simulink model "ASM_Traffic_A11"  (R2026a)
settings: Solver=ode1  StartTime=SIM.tstart.v  StopTime=SIM.tend.v  FixedStep=SIM.StepSize.v
PostLoadFcn:
  | if any(exist('dsrtsu_mdlpostloadfcn', 'file') ~= 0), dsrtsu_mdlpostloadfcn('Execute', bdroot); end
  | try, asm_mdl_postloadfcn(bdroot, 'UpdateModel', 3600); catch, disp(lasterr); end,
InitFcn:
  | , if any(exist('rtifpga_mdlclblib', 'file') ~= 0), rtifpga_mdlclblib('Init', bdroot); end,
  | , if any(exist('dsmpb_private', 'file') ~= 0), dsmpb_private('dsmpb_mdlclblib', 'Init', bdroot); end,
undefined symbols (not defined in the file): _to_, a0b2, ASM_BrakeHydraulics_DemoSystems, ASM_VehicleDynamics_DemoSystems, b98103fe8ad365046cd0, BrakeCircuit, controllerConfig, CPT, Crankshaft, DiscIntNeverNeededParam, dsmsi, FinalDriveAssembly, instance, MDL, ModeSignals, mu, Pos_BrakePedal_Maneuver, rad, RefSignals, s_to_rpm, SIM, SoftECU, Suspension, Tire, Transmission
libraries: ASM_Traffic_lib x135, simulink x98, ASM_Utils_lib x77, ASM_VehicleDynamics_lib x70, ASM_Environment_lib x22, dsmpblib x20, dsmsilib x15, MDLD_Utils_lib x10, ASM_BrakeHydraulics_lib x3, sl_discontinuities x2
(part 62 of 63)

== system ASM_Traffic_A11/Environment/Sensors/PlantModel/Object_Sensor_3D/ObjectData/Sensor1/Object_Custom_Values/Vectorize_Signals ==
  SensorOutput1 : Inport
  SensorOutput2 : Inport  Port=2
  SensorOutput3 : Inport  Port=3
  Bus Creator : BusCreator  Inputs=2
  Bus Selector : BusSelector  OutputSignals=SensorOutput.Object1.Object_Valid[0|1],SensorOutput.Object2.Object_Valid[0|1],SensorOutput.Object3.Object_Valid[0|1],SensorOutput.Object4.Object_Valid[0|1],SensorOutput.Object5.Object_Valid[0|1]
  Bus Selector1 : BusSelector  OutputSignals=SensorOutput.Object1.Object_Valid[0|1],SensorOutput.Object2.Object_Valid[0|1],SensorOutput.Object3.Object_Valid[0|1],SensorOutput.Object4.Object_Valid[0|1],SensorOutput.Object5.Object_Valid[0|1]
  Bus Selector2 : BusSelector  OutputSignals=SensorOutput.Object1.Object_Valid[0|1],SensorOutput.Object2.Object_Valid[0|1],SensorOutput.Object3.Object_Valid[0|1],SensorOutput.Object4.Object_Valid[0|1],SensorOutput.Object5.Object_Valid[0|1]
  Bus Selector3 : BusSelector  OutputSignals=SensorOutput.Object1.CustomValues[],SensorOutput.Object2.CustomValues[],SensorOutput.Object3.CustomValues[],SensorOutput.Object4.CustomValues[],SensorOutput.Object5.CustomValues[]
  Bus Selector4 : BusSelector  OutputSignals=SensorOutput.Object1.CustomValues[],SensorOutput.Object2.CustomValues[],SensorOutput.Object3.CustomValues[],SensorOutput.Object4.CustomValues[],SensorOutput.Object5.CustomValues[]
  Bus Selector5 : BusSelector  OutputSignals=SensorOutput.Object1.CustomValues[],SensorOutput.Object2.CustomValues[],SensorOutput.Object3.CustomValues[],SensorOutput.Object4.CustomValues[],SensorOutput.Object5.CustomValues[]
  Mux : Mux  Inputs=15
  Mux1 : Mux  Inputs=15
  Vectorized_Custom_Values : Outport  VectorParamsAs1DForOutWhenUnconnected=off
  wires:
  Bus Creator/1 -> Vectorized_Custom_Values/1
  Bus Selector5/5 -> Mux1/15  "<CustomValues[]>"
  Bus Selector5/4 -> Mux1/14  "<CustomValues[]>"
  Bus Selector5/3 -> Mux1/13  "<CustomValues[]>"
  Bus Selector5/2 -> Mux1/12  "<CustomValues[]>"
  Bus Selector5/1 -> Mux1/11  "<CustomValues[]>"
  Bus Selector4/5 -> Mux1/10  "<CustomValues[]>"
  Bus Selector4/4 -> Mux1/9  "<CustomValues[]>"
  Bus Selector4/3 -> Mux1/8  "<CustomValues[]>"
  Bus Selector4/2 -> Mux1/7  "<CustomValues[]>"
  Bus Selector4/1 -> Mux1/6  "<CustomValues[]>"
  Bus Selector3/5 -> Mux1/5  "<CustomValues[]>"
  Bus Selector3/4 -> Mux1/4  "<CustomValues[]>"
  Bus Selector3/3 -> Mux1/3  "<CustomValues[]>"
  Bus Selector3/2 -> Mux1/2  "<CustomValues[]>"
  Bus Selector3/1 -> Mux1/1  "<CustomValues[]>"
  Bus Selector2/5 -> Mux/15  "<Object_Valid[0|1]>"
  Bus Selector2/4 -> Mux/14  "<Object_Valid[0|1]>"
  Bus Selector2/3 -> Mux/13  "<Object_Valid[0|1]>"
  Bus Selector2/2 -> Mux/12  "<Object_Valid[0|1]>"
  Bus Selector2/1 -> Mux/11  "<Object_Valid[0|1]>"
  Bus Selector1/5 -> Mux/10  "<Object_Valid[0|1]>"
  Bus Selector1/4 -> Mux/9  "<Object_Valid[0|1]>"
  Bus Selector1/3 -> Mux/8  "<Object_Valid[0|1]>"
  Bus Selector1/2 -> Mux/7  "<Object_Valid[0|1]>"
  Bus Selector1/1 -> Mux/6  "<Object_Valid[0|1]>"
  Mux1/1 -> Bus Creator/2  "CustomValues[]"
  Mux/1 -> Bus Creator/1  "Object_Valid[0|1]"
  SensorOutput3/1 -> Bus Selector2/1, Bus Selector5/1
  SensorOutput2/1 -> Bus Selector1/1, Bus Selector4/1
  Bus Selector/1 -> Mux/1  "<Object_Valid[0|1]>"
  Bus Selector/2 -> Mux/2  "<Object_Valid[0|1]>"
  Bus Selector/3 -> Mux/3  "<Object_Valid[0|1]>"
  Bus Selector/4 -> Mux/4  "<Object_Valid[0|1]>"
  Bus Selector/5 -> Mux/5  "<Object_Valid[0|1]>"
  SensorOutput1/1 -> Bus Selector3/1, Bus Selector/1

== system ASM_Traffic_A11/Environment/Sensors/PlantModel/Object_Sensor_3D/ObjectData/Sensor2/Object_Custom_Values/Vectorize_Signals ==
  SensorOutput1 : Inport
  SensorOutput2 : Inport  Port=2
  SensorOutput3 : Inport  Port=3
  Bus Creator : BusCreator  Inputs=2
  Bus Selector : BusSelector  OutputSignals=SensorOutput.Object1.Object_Valid[0|1],SensorOutput.Object2.Object_Valid[0|1],SensorOutput.Object3.Object_Valid[0|1],SensorOutput.Object4.Object_Valid[0|1],SensorOutput.Object5.Object_Valid[0|1]
  Bus Selector1 : BusSelector  OutputSignals=SensorOutput.Object1.Object_Valid[0|1],SensorOutput.Object2.Object_Valid[0|1],SensorOutput.Object3.Object_Valid[0|1],SensorOutput.Object4.Object_Valid[0|1],SensorOutput.Object5.Object_Valid[0|1]
  Bus Selector2 : BusSelector  OutputSignals=SensorOutput.Object1.Object_Valid[0|1],SensorOutput.Object2.Object_Valid[0|1],SensorOutput.Object3.Object_Valid[0|1],SensorOutput.Object4.Object_Valid[0|1],SensorOutput.Object5.Object_Valid[0|1]
  Bus Selector3 : BusSelector  OutputSignals=SensorOutput.Object1.CustomValues[],SensorOutput.Object2.CustomValues[],SensorOutput.Object3.CustomValues[],SensorOutput.Object4.CustomValues[],SensorOutput.Object5.CustomValues[]
  Bus Selector4 : BusSelector  OutputSignals=SensorOutput.Object1.CustomValues[],SensorOutput.Object2.CustomValues[],SensorOutput.Object3.CustomValues[],SensorOutput.Object4.CustomValues[],SensorOutput.Object5.CustomValues[]
  Bus Selector5 : BusSelector  OutputSignals=SensorOutput.Object1.CustomValues[],SensorOutput.Object2.CustomValues[],SensorOutput.Object3.CustomValues[],SensorOutput.Object4.CustomValues[],SensorOutput.Object5.CustomValues[]
  Mux : Mux  Inputs=15
  Mux1 : Mux  Inputs=15
  Vectorized_Custom_Values : Outport  VectorParamsAs1DForOutWhenUnconnected=off
  wires:
  SensorOutput1/1 -> Bus Selector/1, Bus Selector3/1
  Bus Selector/5 -> Mux/5  "<Object_Valid[0|1]>"
  Bus Selector/4 -> Mux/4  "<Object_Valid[0|1]>"
  Bus Selector/3 -> Mux/3  "<Object_Valid[0|1]>"
  Bus Selector/2 -> Mux/2  "<Object_Valid[0|1]>"
  Bus Selector/1 -> Mux/1  "<Object_Valid[0|1]>"
  SensorOutput2/1 -> Bus Selector4/1, Bus Selector1/1
  SensorOutput3/1 -> Bus Selector5/1, Bus Selector2/1
  Mux/1 -> Bus Creator/1  "Object_Valid[0|1]"
  Mux1/1 -> Bus Creator/2  "CustomValues[]"
  Bus Selector1/1 -> Mux/6  "<Object_Valid[0|1]>"
  Bus Selector1/2 -> Mux/7  "<Object_Valid[0|1]>"
  Bus Selector1/3 -> Mux/8  "<Object_Valid[0|1]>"
  Bus Selector1/4 -> Mux/9  "<Object_Valid[0|1]>"
  Bus Selector1/5 -> Mux/10  "<Object_Valid[0|1]>"
  Bus Selector2/1 -> Mux/11  "<Object_Valid[0|1]>"
  Bus Selector2/2 -> Mux/12  "<Object_Valid[0|1]>"
  Bus Selector2/3 -> Mux/13  "<Object_Valid[0|1]>"
  Bus Selector2/4 -> Mux/14  "<Object_Valid[0|1]>"
  Bus Selector2/5 -> Mux/15  "<Object_Valid[0|1]>"
  Bus Selector3/1 -> Mux1/1  "<CustomValues[]>"
  Bus Selector3/2 -> Mux1/2  "<CustomValues[]>"
  Bus Selector3/3 -> Mux1/3  "<CustomValues[]>"
  Bus Selector3/4 -> Mux1/4  "<CustomValues[]>"
  Bus Selector3/5 -> Mux1/5  "<CustomValues[]>"
  Bus Selector4/1 -> Mux1/6  "<CustomValues[]>"
  Bus Selector4/2 -> Mux1/7  "<CustomValues[]>"
  Bus Selector4/3 -> Mux1/8  "<CustomValues[]>"
  Bus Selector4/4 -> Mux1/9  "<CustomValues[]>"
  Bus Selector4/5 -> Mux1/10  "<CustomValues[]>"
  Bus Selector5/1 -> Mux1/11  "<CustomValues[]>"
  Bus Selector5/2 -> Mux1/12  "<CustomValues[]>"
  Bus Selector5/3 -> Mux1/13  "<CustomValues[]>"
  Bus Selector5/4 -> Mux1/14  "<CustomValues[]>"
  Bus Selector5/5 -> Mux1/15  "<CustomValues[]>"
  Bus Creator/1 -> Vectorized_Custom_Values/1

== system ASM_Traffic_A11/Environment/Sensors/PlantModel/Object_Sensor_3D/ObjectData/Sensor3/Object_Custom_Values/Vectorize_Signals ==
  SensorOutput1 : Inport
  SensorOutput2 : Inport  Port=2
  SensorOutput3 : Inport  Port=3
  Bus Creator : BusCreator  Inputs=2
  Bus Selector : BusSelector  OutputSignals=SensorOutput.Object1.Object_Valid[0|1],SensorOutput.Object2.Object_Valid[0|1],SensorOutput.Object3.Object_Valid[0|1],SensorOutput.Object4.Object_Valid[0|1],SensorOutput.Object5.Object_Valid[0|1]
  Bus Selector1 : BusSelector  OutputSignals=SensorOutput.Object1.Object_Valid[0|1],SensorOutput.Object2.Object_Valid[0|1],SensorOutput.Object3.Object_Valid[0|1],SensorOutput.Object4.Object_Valid[0|1],SensorOutput.Object5.Object_Valid[0|1]
  Bus Selector2 : BusSelector  OutputSignals=SensorOutput.Object1.Object_Valid[0|1],SensorOutput.Object2.Object_Valid[0|1],SensorOutput.Object3.Object_Valid[0|1],SensorOutput.Object4.Object_Valid[0|1],SensorOutput.Object5.Object_Valid[0|1]
  Bus Selector3 : BusSelector  OutputSignals=SensorOutput.Object1.CustomValues[],SensorOutput.Object2.CustomValues[],SensorOutput.Object3.CustomValues[],SensorOutput.Object4.CustomValues[],SensorOutput.Object5.CustomValues[]
  Bus Selector4 : BusSelector  OutputSignals=SensorOutput.Object1.CustomValues[],SensorOutput.Object2.CustomValues[],SensorOutput.Object3.CustomValues[],SensorOutput.Object4.CustomValues[],SensorOutput.Object5.CustomValues[]
  Bus Selector5 : BusSelector  OutputSignals=SensorOutput.Object1.CustomValues[],SensorOutput.Object2.CustomValues[],SensorOutput.Object3.CustomValues[],SensorOutput.Object4.CustomValues[],SensorOutput.Object5.CustomValues[]
  Mux : Mux  Inputs=15
  Mux1 : Mux  Inputs=15
  Vectorized_Custom_Values : Outport  VectorParamsAs1DForOutWhenUnconnected=off
  wires:
  Bus Creator/1 -> Vectorized_Custom_Values/1
  Bus Selector5/5 -> Mux1/15  "<CustomValues[]>"
  Bus Selector5/4 -> Mux1/14  "<CustomValues[]>"
  Bus Selector5/3 -> Mux1/13  "<CustomValues[]>"
  Bus Selector5/2 -> Mux1/12  "<CustomValues[]>"
  Bus Selector5/1 -> Mux1/11  "<CustomValues[]>"
  Bus Selector4/5 -> Mux1/10  "<CustomValues[]>"
  Bus Selector4/4 -> Mux1/9  "<CustomValues[]>"
  Bus Selector4/3 -> Mux1/8  "<CustomValues[]>"
  Bus Selector4/2 -> Mux1/7  "<CustomValues[]>"
  Bus Selector4/1 -> Mux1/6  "<CustomValues[]>"
  Bus Selector3/5 -> Mux1/5  "<CustomValues[]>"
  Bus Selector3/4 -> Mux1/4  "<CustomValues[]>"
  Bus Selector3/3 -> Mux1/3  "<CustomValues[]>"
  Bus Selector3/2 -> Mux1/2  "<CustomValues[]>"
  Bus Selector3/1 -> Mux1/1  "<CustomValues[]>"
  Bus Selector2/5 -> Mux/15  "<Object_Valid[0|1]>"
  Bus Selector2/4 -> Mux/14  "<Object_Valid[0|1]>"
  Bus Selector2/3 -> Mux/13  "<Object_Valid[0|1]>"
  Bus Selector2/2 -> Mux/12  "<Object_Valid[0|1]>"
  Bus Selector2/1 -> Mux/11  "<Object_Valid[0|1]>"
  Bus Selector1/5 -> Mux/10  "<Object_Valid[0|1]>"
  Bus Selector1/4 -> Mux/9  "<Object_Valid[0|1]>"
  Bus Selector1/3 -> Mux/8  "<Object_Valid[0|1]>"
  Bus Selector1/2 -> Mux/7  "<Object_Valid[0|1]>"
  Bus Selector1/1 -> Mux/6  "<Object_Valid[0|1]>"
  Mux1/1 -> Bus Creator/2  "CustomValues[]"
  Mux/1 -> Bus Creator/1  "Object_Valid[0|1]"
  SensorOutput3/1 -> Bus Selector2/1, Bus Selector5/1
  SensorOutput2/1 -> Bus Selector1/1, Bus Selector4/1
  Bus Selector/1 -> Mux/1  "<Object_Valid[0|1]>"
  Bus Selector/2 -> Mux/2  "<Object_Valid[0|1]>"
  Bus Selector/3 -> Mux/3  "<Object_Valid[0|1]>"
  Bus Selector/4 -> Mux/4  "<Object_Valid[0|1]>"
  Bus Selector/5 -> Mux/5  "<Object_Valid[0|1]>"
  SensorOutput1/1 -> Bus Selector3/1, Bus Selector/1

== system ASM_Traffic_A11/Environment/Sensors/PlantModel/Object_Sensor_3D/RadarEffects/Sensor1/RadarEffectsOutput/HoldSignals ==
  ResetPulse[0|1] : Inport
  RadarEffect_Signals_In[] : Inport  Port=2
  Enable : EnablePort
  Bus Selector1 : BusSelector  OutputSignals=ID[],Dist_CoorSys_S[m],v_CoorSys_S[m|s],Angle_Hor_CoorSys_S[deg],Angle_Ver_CoorSys_S[deg],RCS[dBm2],Object_ID[],Object_Type[],Pos_ObjectPoint_CoorSys_E[x;y;z][m],Pos_ObjectPoint_CoorSys_S[x;y;z][m]
  RADAR_SIGNALS_RESET_1 : ASM_Traffic_lib/Sensors/RadarEffects/RADAR_SIGNALS_RESET  ASMProperties=struct('Name','RADAR_SIGNALS_RESET','Version','1.0','Library','ASM_Traffic_lib')  ASMInstanceName=radar_signals_reset  ASMInstanceID=1
  RadarEffect_Signals_Out[] : Outport  VectorParamsAs1DForOutWhenUnconnected=off
  wires:
  ResetPulse[0|1]/1 -> RADAR_SIGNALS_RESET_1/1
  RADAR_SIGNALS_RESET_1/1 -> RadarEffect_Signals_Out[]/1
  Bus Selector1/3 -> RADAR_SIGNALS_RESET_1/4  "<v_CoorSys_S[m|s]>"
  Bus Selector1/2 -> RADAR_SIGNALS_RESET_1/3  "<Dist_CoorSys_S[m]>"
  Bus Selector1/7 -> RADAR_SIGNALS_RESET_1/8  "<Object_ID[]>"
  Bus Selector1/6 -> RADAR_SIGNALS_RESET_1/7  "<RCS[dBm2]>"
  Bus Selector1/4 -> RADAR_SIGNALS_RESET_1/5  "<Angle_Hor_CoorSys_S[deg]>"
  Bus Selector1/1 -> RADAR_SIGNALS_RESET_1/2  "<ID[]>"
  Bus Selector1/9 -> RADAR_SIGNALS_RESET_1/10  "<Pos_ObjectPoint_CoorSys_E[x;y;z][m]>"
  Bus Selector1/5 -> RADAR_SIGNALS_RESET_1/6  "<Angle_Ver_CoorSys_S[deg]>"
  Bus Selector1/8 -> RADAR_SIGNALS_RESET_1/9  "<Object_Type[]>"
  Bus Selector1/10 -> RADAR_SIGNALS_RESET_1/11  "<Pos_ObjectPoint_CoorSys_S[x;y;z][m]>"
  RadarEffect_Signals_In[]/1 -> Bus Selector1/1

== system ASM_Traffic_A11/Environment/Sensors/PlantModel/Object_Sensor_3D/RadarEffects/Sensor1/RadarEffectsOutput/ResetPulse ==
  Enable[0|1] : Inport
  SensorActive[0|1] : Inport  Port=2
  Compare To Constant : simulink/Logic and Bit Operations/Compare To Constant  relop===  const=1  OutDataTypeStr=boolean
  Compare To Constant1 : simulink/Logic and Bit Operations/Compare To Constant  relop===  const=0  OutDataTypeStr=boolean
  Logical Operator1 : Logic  AllPortsSameDT=off  OutDataTypeStr=boolean
  Logical Operator2 : Logic  Operator=NAND  AllPortsSameDT=off  OutDataTypeStr=boolean
  Memory1 : UnitDelay  SampleTime=-1
  ResetPulse[0|1] : Outport  VectorParamsAs1DForOutWhenUnconnected=off
  wires:
  Memory1/1 -> Compare To Constant1/1
  Logical Operator2/1 -> Compare To Constant/1, Memory1/1
  SensorActive[0|1]/1 -> Logical Operator2/1
  Logical Operator1/1 -> ResetPulse[0|1]/1
  Compare To Constant/1 -> Logical Operator1/1
  Compare To Constant1/1 -> Logical Operator1/2
  Enable[0|1]/1 -> Logical Operator2/2

== system ASM_Traffic_A11/Environment/Sensors/PlantModel/Object_Sensor_3D/RadarEffects/Sensor1/RadarEffectsOutput/SignalBus ==
  RadarEffect_Signals_In[] : Inport
  Bus Creator : BusCreator  Inputs=5
  Bus Selector1 : BusSelector  OutputSignals=ID[],Object_ID[],Dist_CoorSys_S[m],Angle_Hor_CoorSys_S[deg],Pos_ObjectPoint_CoorSys_E[x;y;z][m]
  RadarEffect_Signals_Out[] : Outport  VectorParamsAs1DForOutWhenUnconnected=off
  wires:
  RadarEffect_Signals_In[]/1 -> Bus Selector1/1
  Bus Creator/1 -> RadarEffect_Signals_Out[]/1
  Bus Selector1/4 -> Bus Creator/4  "<Angle_Hor_CoorSys_S[deg]>"
  Bus Selector1/5 -> Bus Creator/5  "<Pos_ObjectPoint_CoorSys_E[x;y;z][m]>"
  Bus Selector1/2 -> Bus Creator/2  "<Object_ID[]>"
  Bus Selector1/3 -> Bus Creator/3  "<Dist_CoorSys_S[m]>"
  Bus Selector1/1 -> Bus Creator/1  "<ID[]>"

== system ASM_Traffic_A11/Environment/Sensors/PlantModel/Object_Sensor_3D/RadarEffects/Sensor2/RadarEffectsOutput/HoldSignals ==
  ResetPulse[0|1] : Inport
  RadarEffect_Signals_In[] : Inport  Port=2
  Enable : EnablePort
  Bus Selector1 : BusSelector  OutputSignals=ID[],Dist_CoorSys_S[m],v_CoorSys_S[m|s],Angle_Hor_CoorSys_S[deg],Angle_Ver_CoorSys_S[deg],RCS[dBm2],Object_ID[],Object_Type[],Pos_ObjectPoint_CoorSys_E[x;y;z][m],Pos_ObjectPoint_CoorSys_S[x;y;z][m]
  RADAR_SIGNALS_RESET_2 : ASM_Traffic_lib/Sensors/RadarEffects/RADAR_SIGNALS_RESET  ASMProperties=struct('Name','RADAR_SIGNALS_RESET','Version','1.0','Library','ASM_Traffic_lib')  ASMInstanceName=radar_signals_reset  ASMInstanceID=1
  RadarEffect_Signals_Out[] : Outport  VectorParamsAs1DForOutWhenUnconnected=off
  wires:
  ResetPulse[0|1]/1 -> RADAR_SIGNALS_RESET_2/1
  Bus Selector1/8 -> RADAR_SIGNALS_RESET_2/9  "<Object_Type[]>"
  Bus Selector1/3 -> RADAR_SIGNALS_RESET_2/4  "<v_CoorSys_S[m|s]>"
  Bus Selector1/7 -> RADAR_SIGNALS_RESET_2/8  "<Object_ID[]>"
  RadarEffect_Signals_In[]/1 -> Bus Selector1/1
  Bus Selector1/6 -> RADAR_SIGNALS_RESET_2/7  "<RCS[dBm2]>"
  Bus Selector1/5 -> RADAR_SIGNALS_RESET_2/6  "<Angle_Ver_CoorSys_S[deg]>"
  Bus Selector1/4 -> RADAR_SIGNALS_RESET_2/5  "<Angle_Hor_CoorSys_S[deg]>"
  Bus Selector1/2 -> RADAR_SIGNALS_RESET_2/3  "<Dist_CoorSys_S[m]>"
  Bus Selector1/10 -> RADAR_SIGNALS_RESET_2/11  "<Pos_ObjectPoint_CoorSys_S[x;y;z][m]>"
  Bus Selector1/1 -> RADAR_SIGNALS_RESET_2/2  "<ID[]>"
  Bus Selector1/9 -> RADAR_SIGNALS_RESET_2/10  "<Pos_ObjectPoint_CoorSys_E[x;y;z][m]>"
  RADAR_SIGNALS_RESET_2/1 -> RadarEffect_Signals_Out[]/1

== system ASM_Traffic_A11/Environment/Sensors/PlantModel/Object_Sensor_3D/RadarEffects/Sensor2/RadarEffectsOutput/ResetPulse ==
  Enable[0|1] : Inport
  SensorActive[0|1] : Inport  Port=2
  Compare To Constant : simulink/Logic and Bit Operations/Compare To Constant  relop===  const=1  OutDataTypeStr=boolean
  Compare To Constant1 : simulink/Logic and Bit Operations/Compare To Constant  relop===  const=0  OutDataTypeStr=boolean
  Logical Operator1 : Logic  AllPortsSameDT=off  OutDataTypeStr=boolean
  Logical Operator2 : Logic  Operator=NAND  AllPortsSameDT=off  OutDataTypeStr=boolean
  Memory1 : UnitDelay  SampleTime=-1
  ResetPulse[0|1] : Outport  VectorParamsAs1DForOutWhenUnconnected=off
  wires:
  Memory1/1 -> Compare To Constant1/1
  Logical Operator2/1 -> Compare To Constant/1, Memory1/1
  SensorActive[0|1]/1 -> Logical Operator2/1
  Logical Operator1/1 -> ResetPulse[0|1]/1
  Compare To Constant/1 -> Logical Operator1/1
  Compare To Constant1/1 -> Logical Operator1/2
  Enable[0|1]/1 -> Logical Operator2/2

== system ASM_Traffic_A11/Environment/Sensors/PlantModel/Object_Sensor_3D/RadarEffects/Sensor2/RadarEffectsOutput/SignalBus ==
  RadarEffect_Signals_In[] : Inport
  Bus Creator : BusCreator  Inputs=5
  Bus Selector1 : BusSelector  OutputSignals=ID[],Object_ID[],Dist_CoorSys_S[m],Angle_Hor_CoorSys_S[deg],Pos_ObjectPoint_CoorSys_E[x;y;z][m]
  RadarEffect_Signals_Out[] : Outport  VectorParamsAs1DForOutWhenUnconnected=off
  wires:
  RadarEffect_Signals_In[]/1 -> Bus Selector1/1
  Bus Creator/1 -> RadarEffect_Signals_Out[]/1
  Bus Selector1/4 -> Bus Creator/4  "<Angle_Hor_CoorSys_S[deg]>"
  Bus Selector1/5 -> Bus Creator/5  "<Pos_ObjectPoint_CoorSys_E[x;y;z][m]>"
  Bus Selector1/2 -> Bus Creator/2  "<Object_ID[]>"
  Bus Selector1/3 -> Bus Creator/3  "<Dist_CoorSys_S[m]>"
  Bus Selector1/1 -> Bus Creator/1  "<ID[]>"

== system ASM_Traffic_A11/Environment/Sensors/PlantModel/Object_Sensor_3D/RadarEffects/Sensor3/RadarEffectsOutput/HoldSignals ==
  ResetPulse[0|1] : Inport
  RadarEffect_Signals_In[] : Inport  Port=2
  Enable : EnablePort
  Bus Selector1 : BusSelector  OutputSignals=ID[],Dist_CoorSys_S[m],v_CoorSys_S[m|s],Angle_Hor_CoorSys_S[deg],Angle_Ver_CoorSys_S[deg],RCS[dBm2],Object_ID[],Object_Type[],Pos_ObjectPoint_CoorSys_E[x;y;z][m],Pos_ObjectPoint_CoorSys_S[x;y;z][m]
  RADAR_SIGNALS_RESET_3 : ASM_Traffic_lib/Sensors/RadarEffects/RADAR_SIGNALS_RESET  ASMProperties=struct('Name','RADAR_SIGNALS_RESET','Version','1.0','Library','ASM_Traffic_lib')  ASMInstanceName=radar_signals_reset  ASMInstanceID=1
  RadarEffect_Signals_Out[] : Outport  VectorParamsAs1DForOutWhenUnconnected=off
  wires:
  RADAR_SIGNALS_RESET_3/1 -> RadarEffect_Signals_Out[]/1
  Bus Selector1/9 -> RADAR_SIGNALS_RESET_3/10  "<Pos_ObjectPoint_CoorSys_E[x;y;z][m]>"
  Bus Selector1/5 -> RADAR_SIGNALS_RESET_3/6  "<Angle_Ver_CoorSys_S[deg]>"
  Bus Selector1/4 -> RADAR_SIGNALS_RESET_3/5  "<Angle_Hor_CoorSys_S[deg]>"
  Bus Selector1/1 -> RADAR_SIGNALS_RESET_3/2  "<ID[]>"
  ResetPulse[0|1]/1 -> RADAR_SIGNALS_RESET_3/1
  Bus Selector1/6 -> RADAR_SIGNALS_RESET_3/7  "<RCS[dBm2]>"
  Bus Selector1/7 -> RADAR_SIGNALS_RESET_3/8  "<Object_ID[]>"
  Bus Selector1/3 -> RADAR_SIGNALS_RESET_3/4  "<v_CoorSys_S[m|s]>"
  RadarEffect_Signals_In[]/1 -> Bus Selector1/1
  Bus Selector1/10 -> RADAR_SIGNALS_RESET_3/11  "<Pos_ObjectPoint_CoorSys_S[x;y;z][m]>"
  Bus Selector1/8 -> RADAR_SIGNALS_RESET_3/9  "<Object_Type[]>"
  Bus Selector1/2 -> RADAR_SIGNALS_RESET_3/3  "<Dist_CoorSys_S[m]>"

== system ASM_Traffic_A11/Environment/Sensors/PlantModel/Object_Sensor_3D/RadarEffects/Sensor3/RadarEffectsOutput/ResetPulse ==
  Enable[0|1] : Inport
  SensorActive[0|1] : Inport  Port=2
  Compare To Constant : simulink/Logic and Bit Operations/Compare To Constant  relop===  const=1  OutDataTypeStr=boolean
  Compare To Constant1 : simulink/Logic and Bit Operations/Compare To Constant  relop===  const=0  OutDataTypeStr=boolean
  Logical Operator1 : Logic  AllPortsSameDT=off  OutDataTypeStr=boolean
  Logical Operator2 : Logic  Operator=NAND  AllPortsSameDT=off  OutDataTypeStr=boolean
  Memory1 : UnitDelay  SampleTime=-1
  ResetPulse[0|1] : Outport  VectorParamsAs1DForOutWhenUnconnected=off
  wires:
  Memory1/1 -> Compare To Constant1/1
  Logical Operator2/1 -> Compare To Constant/1, Memory1/1
  SensorActive[0|1]/1 -> Logical Operator2/1
  Logical Operator1/1 -> ResetPulse[0|1]/1
  Compare To Constant/1 -> Logical Operator1/1
  Compare To Constant1/1 -> Logical Operator1/2
  Enable[0|1]/1 -> Logical Operator2/2

== system ASM_Traffic_A11/Environment/Sensors/PlantModel/Object_Sensor_3D/RadarEffects/Sensor3/RadarEffectsOutput/SignalBus ==
  RadarEffect_Signals_In[] : Inport
  Bus Creator : BusCreator  Inputs=5
  Bus Selector1 : BusSelector  OutputSignals=ID[],Object_ID[],Dist_CoorSys_S[m],Angle_Hor_CoorSys_S[deg],Pos_ObjectPoint_CoorSys_E[x;y;z][m]
  RadarEffect_Signals_Out[] : Outport  VectorParamsAs1DForOutWhenUnconnected=off
  wires:
  RadarEffect_Signals_In[]/1 -> Bus Selector1/1
  Bus Creator/1 -> RadarEffect_Signals_Out[]/1
  Bus Selector1/4 -> Bus Creator/4  "<Angle_Hor_CoorSys_S[deg]>"
  Bus Selector1/5 -> Bus Creator/5  "<Pos_ObjectPoint_CoorSys_E[x;y;z][m]>"
  Bus Selector1/2 -> Bus Creator/2  "<Object_ID[]>"
  Bus Selector1/3 -> Bus Creator/3  "<Dist_CoorSys_S[m]>"
  Bus Selector1/1 -> Bus Creator/1  "<ID[]>"

== system ASM_Traffic_A11/Environment/Sensors/UserInterface/DISP_Plant/Object_Sensor_2D/IdxSelect_2DSensor/Scopezone_Element_Data_Selection1/Angle_Hor_Rel[deg]1 ==
  In1 : Inport
  Out1 : Outport  VectorParamsAs1DForOutWhenUnconnected=off
  wires:
  In1/1 -> Out1/1

== system ASM_Traffic_A11/Environment/Sensors/UserInterface/DISP_Plant/Object_Sensor_2D/IdxSelect_2DSensor/Scopezone_Element_Data_Selection1/Distance[m]1 ==
  In1 : Inport
  Out1 : Outport  VectorParamsAs1DForOutWhenUnconnected=off
  wires:
  In1/1 -> Out1/1

== system ASM_Traffic_A11/Environment/Sensors/UserInterface/DISP_Plant/Object_Sensor_2D/IdxSelect_2DSensor/Scopezone_Element_Data_Selection1/Flag_Object_In_Scope[0Out|1In]1 ==
  In1 : Inport
  Out1 : Outport  VectorParamsAs1DForOutWhenUnconnected=off
  wires:
  In1/1 -> Out1/1

== system ASM_Traffic_A11/Environment/Sensors/UserInterface/DISP_Plant/Object_Sensor_2D/IdxSelect_2DSensor/Scopezone_Element_Data_Selection1/Flag_Sensor_Apex_In_Object[0Out|1In]1 ==
  In1 : Inport
  Out1 : Outport  VectorParamsAs1DForOutWhenUnconnected=off
  wires:
  In1/1 -> Out1/1

== system ASM_Traffic_A11/Environment/Sensors/UserInterface/DISP_Plant/Object_Sensor_2D/IdxSelect_2DSensor/Scopezone_Element_Data_Selection1/Height_Max[m]1 ==
  In1 : Inport
  Out1 : Outport  VectorParamsAs1DForOutWhenUnconnected=off
  wires:
  In1/1 -> Out1/1

== system ASM_Traffic_A11/Environment/Sensors/UserInterface/DISP_Plant/Object_Sensor_2D/IdxSelect_2DSensor/Scopezone_Element_Data_Selection1/Height_Min[m]1 ==
  In1 : Inport
  Out1 : Outport  VectorParamsAs1DForOutWhenUnconnected=off
  wires:
  In1/1 -> Out1/1

== system ASM_Traffic_A11/Environment/Sensors/UserInterface/DISP_Plant/Object_Sensor_2D/IdxSelect_2DSensor/Scopezone_Element_Data_Selection1/Object_ID[]1 ==
  In1 : Inport
  Out1 : Outport  VectorParamsAs1DForOutWhenUnconnected=off
  wires:
  In1/1 -> Out1/1

== system ASM_Traffic_A11/Environment/Sensors/UserInterface/DISP_Plant/Object_Sensor_2D/IdxSelect_2DSensor/Scopezone_Element_Data_Selection1/Object_Type[]1 ==
  In1 : Inport
  Out1 : Outport  VectorParamsAs1DForOutWhenUnconnected=off
  wires:
  In1/1 -> Out1/1

== system ASM_Traffic_A11/Environment/Sensors/UserInterface/DISP_Plant/Object_Sensor_2D/IdxSelect_2DSensor/Scopezone_Element_Data_Selection1/a_Rel[m|s2]1 ==
  In1 : Inport
  Out1 : Outport  VectorParamsAs1DForOutWhenUnconnected=off
  wires:
  In1/1 -> Out1/1

== system ASM_Traffic_A11/Environment/Sensors/UserInterface/DISP_Plant/Object_Sensor_2D/IdxSelect_2DSensor/Scopezone_Element_Data_Selection1/v_Rel[m|s]1 ==
  In1 : Inport
  Out1 : Outport  VectorParamsAs1DForOutWhenUnconnected=off
  wires:
  In1/1 -> Out1/1

== system ASM_Traffic_A11/Environment/Sensors/UserInterface/DISP_Plant/Object_Sensor_2D/IdxSelect_2DSensor/Scopezone_Element_Data_Selection2/Angle_Hor_Rel[deg]1 ==
  In1 : Inport
  Out1 : Outport  VectorParamsAs1DForOutWhenUnconnected=off
  wires:
  In1/1 -> Out1/1

== system ASM_Traffic_A11/Environment/Sensors/UserInterface/DISP_Plant/Object_Sensor_2D/IdxSelect_2DSensor/Scopezone_Element_Data_Selection2/Distance[m]1 ==
  In1 : Inport
  Out1 : Outport  VectorParamsAs1DForOutWhenUnconnected=off
  wires:
  In1/1 -> Out1/1

== system ASM_Traffic_A11/Environment/Sensors/UserInterface/DISP_Plant/Object_Sensor_2D/IdxSelect_2DSensor/Scopezone_Element_Data_Selection2/Flag_Object_In_Scope[0Out|1In]1 ==
  In1 : Inport
  Out1 : Outport  VectorParamsAs1DForOutWhenUnconnected=off
  wires:
  In1/1 -> Out1/1

== system ASM_Traffic_A11/Environment/Sensors/UserInterface/DISP_Plant/Object_Sensor_2D/IdxSelect_2DSensor/Scopezone_Element_Data_Selection2/Flag_Sensor_Apex_In_Object[0Out|1In]1 ==
  In1 : Inport
  Out1 : Outport  VectorParamsAs1DForOutWhenUnconnected=off
  wires:
  In1/1 -> Out1/1

== system ASM_Traffic_A11/Environment/Sensors/UserInterface/DISP_Plant/Object_Sensor_2D/IdxSelect_2DSensor/Scopezone_Element_Data_Selection2/Height_Max[m]1 ==
  In1 : Inport
  Out1 : Outport  VectorParamsAs1DForOutWhenUnconnected=off
  wires:
  In1/1 -> Out1/1

== system ASM_Traffic_A11/Environment/Sensors/UserInterface/DISP_Plant/Object_Sensor_2D/IdxSelect_2DSensor/Scopezone_Element_Data_Selection2/Height_Min[m]1 ==
  In1 : Inport
  Out1 : Outport  VectorParamsAs1DForOutWhenUnconnected=off
  wires:
  In1/1 -> Out1/1

== system ASM_Traffic_A11/Environment/Sensors/UserInterface/DISP_Plant/Object_Sensor_2D/IdxSelect_2DSensor/Scopezone_Element_Data_Selection2/Object_ID[]1 ==
  In1 : Inport
  Out1 : Outport  VectorParamsAs1DForOutWhenUnconnected=off
  wires:
  In1/1 -> Out1/1

== system ASM_Traffic_A11/Environment/Sensors/UserInterface/DISP_Plant/Object_Sensor_2D/IdxSelect_2DSensor/Scopezone_Element_Data_Selection2/Object_Type[]1 ==
  In1 : Inport
  Out1 : Outport  VectorParamsAs1DForOutWhenUnconnected=off
  wires:
  In1/1 -> Out1/1

== system ASM_Traffic_A11/Environment/Sensors/UserInterface/DISP_Plant/Object_Sensor_2D/IdxSelect_2DSensor/Scopezone_Element_Data_Selection2/a_Rel[m|s2]1 ==
  In1 : Inport
  Out1 : Outport  VectorParamsAs1DForOutWhenUnconnected=off
  wires:
  In1/1 -> Out1/1

== system ASM_Traffic_A11/Environment/Sensors/UserInterface/DISP_Plant/Object_Sensor_2D/IdxSelect_2DSensor/Scopezone_Element_Data_Selection2/v_Rel[m|s]1 ==
  In1 : Inport
  Out1 : Outport  VectorParamsAs1DForOutWhenUnconnected=off
  wires:
  In1/1 -> Out1/1

== system ASM_Traffic_A11/Environment/Sensors/UserInterface/DISP_Plant/Object_Sensor_2D/IdxSelect_2DSensor/Scopezone_Element_Data_Selection3/Angle_Hor_Rel[deg]1 ==
  In1 : Inport
  Out1 : Outport  VectorParamsAs1DForOutWhenUnconnected=off
  wires:
  In1/1 -> Out1/1

== system ASM_Traffic_A11/Environment/Sensors/UserInterface/DISP_Plant/Object_Sensor_2D/IdxSelect_2DSensor/Scopezone_Element_Data_Selection3/Distance[m]1 ==
  In1 : Inport
  Out1 : Outport  VectorParamsAs1DForOutWhenUnconnected=off
  wires:
  In1/1 -> Out1/1

== system ASM_Traffic_A11/Environment/Sensors/UserInterface/DISP_Plant/Object_Sensor_2D/IdxSelect_2DSensor/Scopezone_Element_Data_Selection3/Flag_Object_In_Scope[0Out|1In]1 ==
  In1 : Inport
  Out1 : Outport  VectorParamsAs1DForOutWhenUnconnected=off
  wires:
  In1/1 -> Out1/1

== system ASM_Traffic_A11/Environment/Sensors/UserInterface/DISP_Plant/Object_Sensor_2D/IdxSelect_2DSensor/Scopezone_Element_Data_Selection3/Flag_Sensor_Apex_In_Object[0Out|1In]1 ==
  In1 : Inport
  Out1 : Outport  VectorParamsAs1DForOutWhenUnconnected=off
  wires:
  In1/1 -> Out1/1

== system ASM_Traffic_A11/Environment/Sensors/UserInterface/DISP_Plant/Object_Sensor_2D/IdxSelect_2DSensor/Scopezone_Element_Data_Selection3/Height_Max[m]1 ==
  In1 : Inport
  Out1 : Outport  VectorParamsAs1DForOutWhenUnconnected=off
  wires:
  In1/1 -> Out1/1

== system ASM_Traffic_A11/Environment/Sensors/UserInterface/DISP_Plant/Object_Sensor_2D/IdxSelect_2DSensor/Scopezone_Element_Data_Selection3/Height_Min[m]1 ==
  In1 : Inport
  Out1 : Outport  VectorParamsAs1DForOutWhenUnconnected=off
  wires:
  In1/1 -> Out1/1

== system ASM_Traffic_A11/Environment/Sensors/UserInterface/DISP_Plant/Object_Sensor_2D/IdxSelect_2DSensor/Scopezone_Element_Data_Selection3/Object_ID[]1 ==
  In1 : Inport
  Out1 : Outport  VectorParamsAs1DForOutWhenUnconnected=off
  wires:
  In1/1 -> Out1/1

== system ASM_Traffic_A11/Environment/Sensors/UserInterface/DISP_Plant/Object_Sensor_2D/IdxSelect_2DSensor/Scopezone_Element_Data_Selection3/Object_Type[]1 ==
  In1 : Inport
  Out1 : Outport  VectorParamsAs1DForOutWhenUnconnected=off
  wires:
  In1/1 -> Out1/1

== system ASM_Traffic_A11/Environment/Sensors/UserInterface/DISP_Plant/Object_Sensor_2D/IdxSelect_2DSensor/Scopezone_Element_Data_Selection3/a_Rel[m|s2]1 ==
  In1 : Inport
  Out1 : Outport  VectorParamsAs1DForOutWhenUnconnected=off
  wires:
  In1/1 -> Out1/1

== system ASM_Traffic_A11/Environment/Sensors/UserInterface/DISP_Plant/Object_Sensor_2D/IdxSelect_2DSensor/Scopezone_Element_Data_Selection3/v_Rel[m|s]1 ==
  In1 : Inport
  Out1 : Outport  VectorParamsAs1DForOutWhenUnconnected=off
  wires:
  In1/1 -> Out1/1

== system ASM_Traffic_A11/Environment/Sensors/UserInterface/DISP_Plant/Object_Sensor_2D/IdxSelect_2DSensor/Scopezone_Element_Data_Selection4/Angle_Hor_Rel[deg]1 ==
  In1 : Inport
  Out1 : Outport  VectorParamsAs1DForOutWhenUnconnected=off
  wires:
  In1/1 -> Out1/1

== system ASM_Traffic_A11/Environment/Sensors/UserInterface/DISP_Plant/Object_Sensor_2D/IdxSelect_2DSensor/Scopezone_Element_Data_Selection4/Distance[m]1 ==
  In1 : Inport
  Out1 : Outport  VectorParamsAs1DForOutWhenUnconnected=off
  wires:
  In1/1 -> Out1/1

== system ASM_Traffic_A11/Environment/Sensors/UserInterface/DISP_Plant/Object_Sensor_2D/IdxSelect_2DSensor/Scopezone_Element_Data_Selection4/Flag_Object_In_Scope[0Out|1In]1 ==
  In1 : Inport
  Out1 : Outport  VectorParamsAs1DForOutWhenUnconnected=off
  wires:
  In1/1 -> Out1/1

== system ASM_Traffic_A11/Environment/Sensors/UserInterface/DISP_Plant/Object_Sensor_2D/IdxSelect_2DSensor/Scopezone_Element_Data_Selection4/Flag_Sensor_Apex_In_Object[0Out|1In]1 ==
  In1 : Inport
  Out1 : Outport  VectorParamsAs1DForOutWhenUnconnected=off
  wires:
  In1/1 -> Out1/1

== system ASM_Traffic_A11/Environment/Sensors/UserInterface/DISP_Plant/Object_Sensor_2D/IdxSelect_2DSensor/Scopezone_Element_Data_Selection4/Height_Max[m]1 ==
  In1 : Inport
  Out1 : Outport  VectorParamsAs1DForOutWhenUnconnected=off
  wires:
  In1/1 -> Out1/1

== system ASM_Traffic_A11/Environment/Sensors/UserInterface/DISP_Plant/Object_Sensor_2D/IdxSelect_2DSensor/Scopezone_Element_Data_Selection4/Height_Min[m]1 ==
  In1 : Inport
  Out1 : Outport  VectorParamsAs1DForOutWhenUnconnected=off
  wires:
  In1/1 -> Out1/1

== system ASM_Traffic_A11/Environment/Sensors/UserInterface/DISP_Plant/Object_Sensor_2D/IdxSelect_2DSensor/Scopezone_Element_Data_Selection4/Object_ID[]1 ==
  In1 : Inport
  Out1 : Outport  VectorParamsAs1DForOutWhenUnconnected=off
  wires:
  In1/1 -> Out1/1

== system ASM_Traffic_A11/Environment/Sensors/UserInterface/DISP_Plant/Object_Sensor_2D/IdxSelect_2DSensor/Scopezone_Element_Data_Selection4/Object_Type[]1 ==
  In1 : Inport
  Out1 : Outport  VectorParamsAs1DForOutWhenUnconnected=off
  wires:
  In1/1 -> Out1/1

== system ASM_Traffic_A11/Environment/Sensors/UserInterface/DISP_Plant/Object_Sensor_2D/IdxSelect_2DSensor/Scopezone_Element_Data_Selection4/a_Rel[m|s2]1 ==
  In1 : Inport
  Out1 : Outport  VectorParamsAs1DForOutWhenUnconnected=off
  wires:
  In1/1 -> Out1/1

== system ASM_Traffic_A11/Environment/Sensors/UserInterface/DISP_Plant/Object_Sensor_2D/IdxSelect_2DSensor/Scopezone_Element_Data_Selection4/v_Rel[m|s]1 ==
  In1 : Inport
  Out1 : Outport  VectorParamsAs1DForOutWhenUnconnected=off
  wires:
  In1/1 -> Out1/1

== system ASM_Traffic_A11/Environment/Sensors/UserInterface/DISP_Plant/Object_Sensor_2D/IdxSelect_2DSensor/Scopezone_Element_Data_Selection5/Angle_Hor_Rel[deg]1 ==
  In1 : Inport
  Out1 : Outport  VectorParamsAs1DForOutWhenUnconnected=off
  wires:
  In1/1 -> Out1/1

== system ASM_Traffic_A11/Environment/Sensors/UserInterface/DISP_Plant/Object_Sensor_2D/IdxSelect_2DSensor/Scopezone_Element_Data_Selection5/Distance[m]1 ==
  In1 : Inport
  Out1 : Outport  VectorParamsAs1DForOutWhenUnconnected=off
  wires:
  In1/1 -> Out1/1

== system ASM_Traffic_A11/Environment/Sensors/UserInterface/DISP_Plant/Object_Sensor_2D/IdxSelect_2DSensor/Scopezone_Element_Data_Selection5/Flag_Object_In_Scope[0Out|1In]1 ==
  In1 : Inport
  Out1 : Outport  VectorParamsAs1DForOutWhenUnconnected=off
  wires:
  In1/1 -> Out1/1

== system ASM_Traffic_A11/Environment/Sensors/UserInterface/DISP_Plant/Object_Sensor_2D/IdxSelect_2DSensor/Scopezone_Element_Data_Selection5/Flag_Sensor_Apex_In_Object[0Out|1In]1 ==
  In1 : Inport
  Out1 : Outport  VectorParamsAs1DForOutWhenUnconnected=off
  wires:
  In1/1 -> Out1/1

== system ASM_Traffic_A11/Environment/Sensors/UserInterface/DISP_Plant/Object_Sensor_2D/IdxSelect_2DSensor/Scopezone_Element_Data_Selection5/Height_Max[m]1 ==
  In1 : Inport
  Out1 : Outport  VectorParamsAs1DForOutWhenUnconnected=off
  wires:
  In1/1 -> Out1/1

== system ASM_Traffic_A11/Environment/Sensors/UserInterface/DISP_Plant/Object_Sensor_2D/IdxSelect_2DSensor/Scopezone_Element_Data_Selection5/Height_Min[m]1 ==
  In1 : Inport
  Out1 : Outport  VectorParamsAs1DForOutWhenUnconnected=off
  wires:
  In1/1 -> Out1/1

== system ASM_Traffic_A11/Environment/Sensors/UserInterface/DISP_Plant/Object_Sensor_2D/IdxSelect_2DSensor/Scopezone_Element_Data_Selection5/Object_ID[]1 ==
  In1 : Inport
  Out1 : Outport  VectorParamsAs1DForOutWhenUnconnected=off
  wires:
  In1/1 -> Out1/1

== system ASM_Traffic_A11/Environment/Sensors/UserInterface/DISP_Plant/Object_Sensor_2D/IdxSelect_2DSensor/Scopezone_Element_Data_Selection5/Object_Type[]1 ==
  In1 : Inport
  Out1 : Outport  VectorParamsAs1DForOutWhenUnconnected=off
  wires:
  In1/1 -> Out1/1

== system ASM_Traffic_A11/Environment/Sensors/UserInterface/DISP_Plant/Object_Sensor_2D/IdxSelect_2DSensor/Scopezone_Element_Data_Selection5/a_Rel[m|s2]1 ==
  In1 : Inport
  Out1 : Outport  VectorParamsAs1DForOutWhenUnconnected=off
  wires:
  In1/1 -> Out1/1

== system ASM_Traffic_A11/Environment/Sensors/UserInterface/DISP_Plant/Object_Sensor_2D/IdxSelect_2DSensor/Scopezone_Element_Data_Selection5/v_Rel[m|s]1 ==
  In1 : Inport
  Out1 : Outport  VectorParamsAs1DForOutWhenUnconnected=off
  wires:
  In1/1 -> Out1/1

== system ASM_Traffic_A11/Environment/Sensors/UserInterface/DISP_Plant/Traffic_Sign_Sensor/GetTrfSgnDataByIndex_1/SwitchObjectPosition/Idx_comp ==
  Idx : Inport
  Add : Sum
  Add1 : Sum  Inputs=+-
  Add2 : Sum
  Add3 : Sum
  Constant : Constant
  Constant1 : Constant
  Constant2 : Constant  Value=2
  Constant3 : Constant  Value=3
  Gain : Gain  Gain=3
  Idx_comp_x : Outport  VectorParamsAs1DForOutWhenUnconnected=off
  Idx_comp_y : Outport  Port=2  VectorParamsAs1DForOutWhenUnconnected=off
  Idx_comp_z : Outport  Port=3  VectorParamsAs1DForOutWhenUnconnected=off
  wires:
  Add3/1 -> Idx_comp_z/1
  Add2/1 -> Idx_comp_y/1
  Constant3/1 -> Add3/2
  Constant2/1 -> Add2/2
  Add/1 -> Idx_comp_x/1
  Gain/1 -> Add/1, Add2/1, Add3/1
  Add1/1 -> Gain/1
  Constant1/1 -> Add1/2
  Idx/1 -> Add1/1
  Constant/1 -> Add/2

== system ASM_Traffic_A11/Environment/Sensors/UserInterface/DISP_Plant/Traffic_Sign_Sensor/GetTrfSgnDataByIndex_1/SwitchObjectPosition/Idx_comp1 ==
  Idx : Inport
  Add : Sum
  Add1 : Sum  Inputs=+-
  Add2 : Sum
  Add3 : Sum
  Constant : Constant
  Constant1 : Constant
  Constant2 : Constant  Value=2
  Constant3 : Constant  Value=3
  Gain : Gain  Gain=3
  Idx_comp_x : Outport  VectorParamsAs1DForOutWhenUnconnected=off
  Idx_comp_y : Outport  Port=2  VectorParamsAs1DForOutWhenUnconnected=off
  Idx_comp_z : Outport  Port=3  VectorParamsAs1DForOutWhenUnconnected=off
  wires:
  Constant/1 -> Add/2
  Idx/1 -> Add1/1
  Constant1/1 -> Add1/2
  Add1/1 -> Gain/1
  Gain/1 -> Add3/1, Add2/1, Add/1
  Add/1 -> Idx_comp_x/1
  Constant2/1 -> Add2/2
  Constant3/1 -> Add3/2
  Add2/1 -> Idx_comp_y/1
  Add3/1 -> Idx_comp_z/1

== system ASM_Traffic_A11/Environment/Sensors/UserInterface/DISP_Plant/Traffic_Sign_Sensor/GetTrfSgnDataByIndex_1/SwitchObjectPosition/Idx_comp2 ==
  Idx : Inport
  Add : Sum
  Add1 : Sum  Inputs=+-
  Add2 : Sum
  Add3 : Sum
  Constant : Constant
  Constant1 : Constant
  Constant2 : Constant  Value=2
  Constant3 : Constant  Value=3
  Gain : Gain  Gain=3
  Idx_comp_x : Outport  VectorParamsAs1DForOutWhenUnconnected=off
  Idx_comp_y : Outport  Port=2  VectorParamsAs1DForOutWhenUnconnected=off
  Idx_comp_z : Outport  Port=3  VectorParamsAs1DForOutWhenUnconnected=off
  wires:
  Add3/1 -> Idx_comp_z/1
  Add2/1 -> Idx_comp_y/1
  Constant3/1 -> Add3/2
  Constant2/1 -> Add2/2
  Add/1 -> Idx_comp_x/1
  Gain/1 -> Add/1, Add2/1, Add3/1
  Add1/1 -> Gain/1
  Constant1/1 -> Add1/2
  Idx/1 -> Add1/1
  Constant/1 -> Add/2

== system ASM_Traffic_A11/Environment/Sensors/UserInterface/DISP_Plant/Traffic_Sign_Sensor/GetTrfSgnDataByIndex_1/SwitchSignProperties/Idx_comp ==
  Idx : Inport
  Add{,2..5} (5 alike) : Sum
  Add1 : Sum  Inputs=+-
  Constant : Constant
  Constant1 : Constant
  Constant2 : Constant  Value=2
  Constant3 : Constant  Value=3
  Constant4 : Constant  Value=4
  Constant5 : Constant  Value=5
  Gain : Gain  Gain=5
  Idx_comp_1 : Outport  VectorParamsAs1DForOutWhenUnconnected=off
  Idx_comp_2 : Outport  Port=2  VectorParamsAs1DForOutWhenUnconnected=off
  Idx_comp_3 : Outport  Port=3  VectorParamsAs1DForOutWhenUnconnected=off
  Idx_comp_4 : Outport  Port=4  VectorParamsAs1DForOutWhenUnconnected=off
  Idx_comp_5 : Outport  Port=5  VectorParamsAs1DForOutWhenUnconnected=off
  wires:
  Add5/1 -> Idx_comp_5/1
  Add4/1 -> Idx_comp_4/1
  Constant5/1 -> Add5/2
  Constant4/1 -> Add4/2
  Gain/1 -> Add/1, Add2/1, Add3/1, Add4/1, Add5/1
  Add3/1 -> Idx_comp_3/1
  Add2/1 -> Idx_comp_2/1
  Constant3/1 -> Add3/2
  Constant2/1 -> Add2/2
  Add/1 -> Idx_comp_1/1
  Add1/1 -> Gain/1
  Constant1/1 -> Add1/2
  Idx/1 -> Add1/1
  Constant/1 -> Add/2

== system ASM_Traffic_A11/Environment/Traffic/UserInterface/DISP_Plant/Fellow_Movement/GetFellowDataByIndex_1/SwitchFellowMovementData/Flag_Fellow_Used[0|1] ==
  In1 : Inport
  Out1 : Outport  VectorParamsAs1DForOutWhenUnconnected=off
  wires:
  In1/1 -> Out1/1

== system ASM_Traffic_A11/Environment/Traffic/UserInterface/DISP_Plant/Fellow_Movement/GetFellowDataByIndex_1/SwitchFellowMovementData/d_Total_Fellow[m] ==
  In1 : Inport
  Out1 : Outport  VectorParamsAs1DForOutWhenUnconnected=off
  wires:
  In1/1 -> Out1/1

== system ASM_Traffic_A11/Environment/Traffic/UserInterface/DISP_Plant/Fellow_Movement/GetFellowDataByIndex_1/SwitchFellowMovementData/s_Fellow[m] ==
  In1 : Inport
  Out1 : Outport  VectorParamsAs1DForOutWhenUnconnected=off
  wires:
  In1/1 -> Out1/1

== system ASM_Traffic_A11/Environment/Traffic/UserInterface/DISP_Plant/Fellow_Movement/GetFellowDataByIndex_1/SwitchFellowMovementData/v_Fellow[km|h] ==
  In1 : Inport
  Out1 : Outport  VectorParamsAs1DForOutWhenUnconnected=off
  wires:
  In1/1 -> Out1/1

== system ASM_Traffic_A11/Environment/Traffic/UserInterface/DISP_Plant/Fellow_Movement/GetFellowDataByIndex_2/SwitchFellowMovementData/Flag_Fellow_Used[0|1] ==
  In1 : Inport
  Out1 : Outport  VectorParamsAs1DForOutWhenUnconnected=off
  wires:
  In1/1 -> Out1/1

== system ASM_Traffic_A11/Environment/Traffic/UserInterface/DISP_Plant/Fellow_Movement/GetFellowDataByIndex_2/SwitchFellowMovementData/d_Total_Fellow[m] ==
  In1 : Inport
  Out1 : Outport  VectorParamsAs1DForOutWhenUnconnected=off
  wires:
  In1/1 -> Out1/1

== system ASM_Traffic_A11/Environment/Traffic/UserInterface/DISP_Plant/Fellow_Movement/GetFellowDataByIndex_2/SwitchFellowMovementData/s_Fellow[m] ==
  In1 : Inport
  Out1 : Outport  VectorParamsAs1DForOutWhenUnconnected=off
  wires:
  In1/1 -> Out1/1

== system ASM_Traffic_A11/Environment/Traffic/UserInterface/DISP_Plant/Fellow_Movement/GetFellowDataByIndex_2/SwitchFellowMovementData/v_Fellow[km|h] ==
  In1 : Inport
  Out1 : Outport  VectorParamsAs1DForOutWhenUnconnected=off
  wires:
  In1/1 -> Out1/1

== system ASM_Traffic_A11/Environment/Traffic/UserInterface/DISP_Plant/Fellow_Movement/GetFellowDataByIndex_3/SwitchFellowMovementData/Flag_Fellow_Used[0|1] ==
  In1 : Inport
  Out1 : Outport  VectorParamsAs1DForOutWhenUnconnected=off
  wires:
  In1/1 -> Out1/1

== system ASM_Traffic_A11/Environment/Traffic/UserInterface/DISP_Plant/Fellow_Movement/GetFellowDataByIndex_3/SwitchFellowMovementData/d_Total_Fellow[m] ==
  In1 : Inport
  Out1 : Outport  VectorParamsAs1DForOutWhenUnconnected=off
  wires:
  In1/1 -> Out1/1

== system ASM_Traffic_A11/Environment/Traffic/UserInterface/DISP_Plant/Fellow_Movement/GetFellowDataByIndex_3/SwitchFellowMovementData/s_Fellow[m] ==
  In1 : Inport
  Out1 : Outport  VectorParamsAs1DForOutWhenUnconnected=off
  wires:
  In1/1 -> Out1/1

== system ASM_Traffic_A11/Environment/Traffic/UserInterface/DISP_Plant/Fellow_Movement/GetFellowDataByIndex_3/SwitchFellowMovementData/v_Fellow[km|h] ==
  In1 : Inport
  Out1 : Outport  VectorParamsAs1DForOutWhenUnconnected=off
  wires:
  In1/1 -> Out1/1

== system ASM_Traffic_A11/VehicleDynamics/Plant/VehicleDynamics/VehicleMovement/ASMSignalCollector/Vehicle_Movement_Info_Car/Accelerations/AbsoluteAcceleration_CoG ==
  v_Vehicle_dt[x;y;z][m|s2] : Inport
  w_Vehicle_dt[x;y;z][rad|s2] : Inport  Port=2
  Pos_i[x;y;z][m] : Inport  Port=3
  a_i_Residual[x;y;z][m|s2] : Inport  Port=4
  Pos_i_dt2[x;y;z][m|s2] : Inport  Port=5
  CROSS_PRODUCT6 : ASM_Utils_lib/MatrixOperations/CROSS_PRODUCT
  Sum4 : Sum  Inputs=++++  SaturateOnIntegerOverflow=on
  a_i[m|s2] : Outport  VectorParamsAs1DForOutWhenUnconnected=off
  wires:
  a_i_Residual[x;y;z][m|s2]/1 -> Sum4/4
  Pos_i_dt2[x;y;z][m|s2]/1 -> Sum4/3
  Pos_i[x;y;z][m]/1 -> CROSS_PRODUCT6/2
  Sum4/1 -> a_i[m|s2]/1
  w_Vehicle_dt[x;y;z][rad|s2]/1 -> CROSS_PRODUCT6/1
  v_Vehicle_dt[x;y;z][m|s2]/1 -> Sum4/1
  CROSS_PRODUCT6/1 -> Sum4/2

== system ASM_Traffic_A11/VehicleDynamics/Plant/VehicleDynamics/VehicleMovement/ASMSignalCollector/Vehicle_Movement_Info_Car/Accelerations/AbsoluteAcceleration_FL ==
  v_Vehicle_dt[x;y;z][m|s2] : Inport
  w_Vehicle_dt[x;y;z][rad|s2] : Inport  Port=2
  Pos_i[x;y;z][m] : Inport  Port=3
  a_i_Residual[x;y;z][m|s2] : Inport  Port=4
  Pos_i_dt2[x;y;z][m|s2] : Inport  Port=5
  CROSS_PRODUCT6 : ASM_Utils_lib/MatrixOperations/CROSS_PRODUCT
  Sum4 : Sum  Inputs=++++  SaturateOnIntegerOverflow=on
  a_i[m|s2] : Outport  VectorParamsAs1DForOutWhenUnconnected=off
  wires:
  a_i_Residual[x;y;z][m|s2]/1 -> Sum4/4
  Pos_i_dt2[x;y;z][m|s2]/1 -> Sum4/3
  Pos_i[x;y;z][m]/1 -> CROSS_PRODUCT6/2
  Sum4/1 -> a_i[m|s2]/1
  w_Vehicle_dt[x;y;z][rad|s2]/1 -> CROSS_PRODUCT6/1
  v_Vehicle_dt[x;y;z][m|s2]/1 -> Sum4/1
  CROSS_PRODUCT6/1 -> Sum4/2

== system ASM_Traffic_A11/VehicleDynamics/Plant/VehicleDynamics/VehicleMovement/ASMSignalCollector/Vehicle_Movement_Info_Car/Accelerations/AbsoluteAcceleration_FR ==
  v_Vehicle_dt[x;y;z][m|s2] : Inport
  w_Vehicle_dt[x;y;z][rad|s2] : Inport  Port=2
  Pos_i[x;y;z][m] : Inport  Port=3
  a_i_Residual[x;y;z][m|s2] : Inport  Port=4
  Pos_i_dt2[x;y;z][m|s2] : Inport  Port=5
  CROSS_PRODUCT6 : ASM_Utils_lib/MatrixOperations/CROSS_PRODUCT
  Sum4 : Sum  Inputs=++++  SaturateOnIntegerOverflow=on
  a_i[m|s2] : Outport  VectorParamsAs1DForOutWhenUnconnected=off
  wires:
  a_i_Residual[x;y;z][m|s2]/1 -> Sum4/4
  Pos_i_dt2[x;y;z][m|s2]/1 -> Sum4/3
  Pos_i[x;y;z][m]/1 -> CROSS_PRODUCT6/2
  Sum4/1 -> a_i[m|s2]/1
  w_Vehicle_dt[x;y;z][rad|s2]/1 -> CROSS_PRODUCT6/1
  v_Vehicle_dt[x;y;z][m|s2]/1 -> Sum4/1
  CROSS_PRODUCT6/1 -> Sum4/2

== system ASM_Traffic_A11/VehicleDynamics/Plant/VehicleDynamics/VehicleMovement/ASMSignalCollector/Vehicle_Movement_Info_Car/Accelerations/AbsoluteAcceleration_RL ==
  v_Vehicle_dt[x;y;z][m|s2] : Inport
  w_Vehicle_dt[x;y;z][rad|s2] : Inport  Port=2
  Pos_i[x;y;z][m] : Inport  Port=3
  a_i_Residual[x;y;z][m|s2] : Inport  Port=4
  Pos_i_dt2[x;y;z][m|s2] : Inport  Port=5
  CROSS_PRODUCT6 : ASM_Utils_lib/MatrixOperations/CROSS_PRODUCT
  Sum4 : Sum  Inputs=++++  SaturateOnIntegerOverflow=on
  a_i[m|s2] : Outport  VectorParamsAs1DForOutWhenUnconnected=off
  wires:
  a_i_Residual[x;y;z][m|s2]/1 -> Sum4/4
  Pos_i_dt2[x;y;z][m|s2]/1 -> Sum4/3
  Pos_i[x;y;z][m]/1 -> CROSS_PRODUCT6/2
  Sum4/1 -> a_i[m|s2]/1
  w_Vehicle_dt[x;y;z][rad|s2]/1 -> CROSS_PRODUCT6/1
  v_Vehicle_dt[x;y;z][m|s2]/1 -> Sum4/1
  CROSS_PRODUCT6/1 -> Sum4/2

== system ASM_Traffic_A11/VehicleDynamics/Plant/VehicleDynamics/VehicleMovement/ASMSignalCollector/Vehicle_Movement_Info_Car/Accelerations/AbsoluteAcceleration_RR ==
  v_Vehicle_dt[x;y;z][m|s2] : Inport
  w_Vehicle_dt[x;y;z][rad|s2] : Inport  Port=2
  Pos_i[x;y;z][m] : Inport  Port=3
  a_i_Residual[x;y;z][m|s2] : Inport  Port=4
  Pos_i_dt2[x;y;z][m|s2] : Inport  Port=5
  CROSS_PRODUCT6 : ASM_Utils_lib/MatrixOperations/CROSS_PRODUCT
  Sum4 : Sum  Inputs=++++  SaturateOnIntegerOverflow=on
  a_i[m|s2] : Outport  VectorParamsAs1DForOutWhenUnconnected=off
  wires:
  a_i_Residual[x;y;z][m|s2]/1 -> Sum4/4
  Pos_i_dt2[x;y;z][m|s2]/1 -> Sum4/3
  Pos_i[x;y;z][m]/1 -> CROSS_PRODUCT6/2
  Sum4/1 -> a_i[m|s2]/1
  w_Vehicle_dt[x;y;z][rad|s2]/1 -> CROSS_PRODUCT6/1
  v_Vehicle_dt[x;y;z][m|s2]/1 -> Sum4/1
  CROSS_PRODUCT6/1 -> Sum4/2
